simulink model "tb_gnc"  (R2026b)
settings: Solver=ode3  StopTime=10  FixedStep=1e-3  EnableMultiTasking=on
values from neighbouring files (symbols this model uses):
  P = F.P    [gnc_fsm_driver.m]    (also in t_gnc_mission.m = r.P; t_t07_gnc_sil.m = shaddad_params('World', 3, 'Assign', false))
  Ts = pr.Ts    [t_gnc_mission.m]
undefined symbols (not defined in the file or in its folder): aligned, DiscIntNeverNeededParam, drive_ready, eul, gnssFixType, headingValid, heartbeat, NavQuality, navValid, pos_W, posStd, power_ready, quality, rc_link_ok, rc_mode_sw, SOC, v_track_meas, valid, vel_B, yawRate
libraries: simulink x3, robotmobilelib x1
settings Model: Creator=aomar  LastModifiedBy=aomar
settings ConfigSet: Description=Shaddad fixed-step 1 ms ode3, multitasking, explicit rate transitions (arch 7, D58).
settings DataIOCC: SignalLogging=off
settings OptimizationCC: SimCompilerOptimization=on
settings DebuggingCC: AlgebraicLoopMsg=error  ArtificialAlgebraicLoopMsg=error  SingleTaskRateTransMsg=error  StrictBusMsg=ErrorOnBusTreatedAsVector
settings SimscapeCC: SimscapeNominalValues="[{\"value\":\"1\",\"unit\":\"A\"},{\"value\":\"1\",\"unit\":\"bar\"},{\"value\":\"1\",\"unit\":\"cm^2\"},{\"value\":\"1\",\"unit\":\"cm^3/s\"},{\"value\":\"1\",\"unit\":\"kJ/kg\"},{\"value\":\"1\",\"unit\":\"kW\"},{\"value\":\"1\",\"unit\":\"l\"},{\"value\":\"1\",\"unit\":\"N\"},{\"value\":\"1\",\"unit\":\"N*m\"},{\"value\":\"1\",\"unit\":\"V\"},{\"value\":\"0.001\",\"unit\":\"Wb\"}]"  SimscapeNormalizeSystem=off  SimscapeUseEnergyAccounting=off

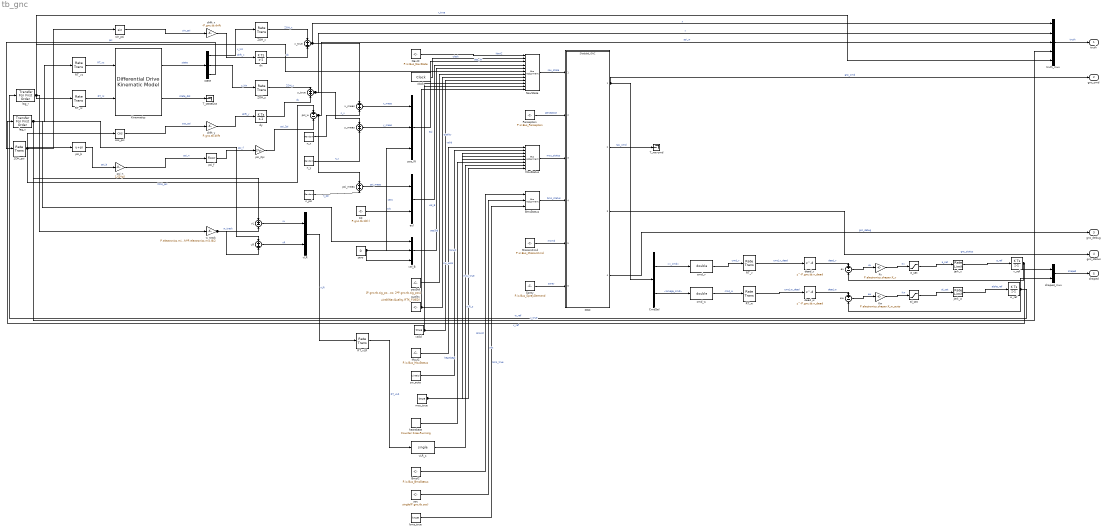
== system tb_gnc ==
  BmsIC : Constant  Value=P.ic.Bus_BmsStatus  OutDataTypeStr=Bus: Bus_BmsStatus  SampleTime=Ts.hk
  BmsStatus : BusAssignment  AssignedSignals=SOC,valid
  CmdSel : BusSelector  OutputSignals=v_cmd,omega_cmd
  GNC : ModelReference  ModelNameDialog=Shaddad_GNC  SimulationMode=Normal  ModelReferenceVersion=1.1
  Kinematics : robotmobilelib/Differential Drive Kinematic Model  VehicleInputs=Vehicle Speed & Heading Angular Velocity  WheelRadius=P.structure.r_sprocket  WheelSpeedRange=[-inf inf]  TrackWidth=P.structure.geom.B  InitialState=P.gnc.tb.x0(:)  SimulateUsing=Code generation
  Kv : Gain  Gain=P.electronics.shaper.K_v
  Kw : Gain  Gain=P.electronics.shaper.K_w_auto
  McuIC : Constant  Value=P.ic.Bus_McuStatus  OutDataTypeStr=Bus: Bus_McuStatus  SampleTime=Ts.gnc
  McuStatus : BusAssignment  AssignedSignals=rc_mode_sw,rc_link_ok,drive_ready,power_ready,heartbeat,v_track_meas,valid
  MissionCmd : Constant  Value=P.ic.Bus_MissionCmd  OutDataTypeStr=Bus: Bus_MissionCmd  SampleTime=Ts.mcmd
  NavIC : Constant  Value=P.ic.Bus_NavState  OutDataTypeStr=Bus: Bus_NavState  SampleTime=Ts.ctrl
  NavState : BusAssignment  AssignedSignals=t,pos_W,eul,vel_B,yawRate,posStd,quality,navValid,headingValid,aligned,gnssFixType
  Perception : Constant  Value=P.ic.Bus_Perception  OutDataTypeStr=Bus: Bus_Perception  SampleTime=Ts.perception
  RT_rc : RateTransition  OutPortSampleTime=0
  RT_v : RateTransition  OutPortSampleTime=Ts.ctrl
  RT_vLR : RateTransition  OutPortSampleTime=Ts.gnc
  RT_vc : RateTransition  OutPortSampleTime=0
  RT_w : RateTransition  OutPortSampleTime=Ts.ctrl
  Spray : Constant  Value=P.ic.Bus_SprayDemand  OutDataTypeStr=Bus: Bus_SprayDemand  SampleTime=Ts.spray
  T_navcmd : Terminator
  T_stateDot : Terminator
  ZOH_psi : RateTransition  OutPortSampleTime=Ts.ctrl
  ZOH_x : RateTransition  OutPortSampleTime=Ts.ctrl
  ZOH_y : RateTransition  OutPortSampleTime=Ts.ctrl
  a_sat : Saturate  UpperLimit=P.electronics.shaper.a_acc_auto  LowerLimit=-P.electronics.shaper.a_dec_auto
  al_sat : Saturate  UpperLimit=P.electronics.shaper.alpha_auto  LowerLimit=-P.electronics.shaper.alpha_auto
  bms_true : Constant  Value=true  OutDataTypeStr=boolean  SampleTime=Ts.hk
  clock : DigitalClock  SampleTime=Ts.ctrl
  cmd_v : DataTypeConversion  OutDataTypeStr=double  SaturateOnIntegerOverflow=off  RndMeth=Floor
  cmd_w : DataTypeConversion  OutDataTypeStr=double  SaturateOnIntegerOverflow=off  RndMeth=Floor
  cos_psi : Trigonometry  Operator=cos
  dead_v : Delay  DelayLength=P.gnc.tb.n_dead  InitialCondition=0  SampleTime=Ts.ctrl
  dead_w : Delay  DelayLength=P.gnc.tb.n_dead  InitialCondition=0  SampleTime=Ts.ctrl
  drift_x : Gain  Gain=-P.gnc.tb.drift
  drift_y : Gain  Gain=P.gnc.tb.drift
  dx : DiscreteIntegrator  SampleTime=Ts.ctrl  ICPrevOutput=DiscIntNeverNeededParam  ICPrevScaledInput=DiscIntNeverNeededParam
  dy : DiscreteIntegrator  SampleTime=Ts.ctrl  ICPrevOutput=DiscIntNeverNeededParam  ICPrevScaledInput=DiscIntNeverNeededParam
  eul : Mux  Inputs=[1 2]
  ev : Sum  Inputs=+-
  ew : Sum  Inputs=+-
  heartbeat : simulink/Sources/Counter Free-Running  NumBits=8  tsamp=Ts.gnc
  jerk_v : RateLimiter  RisingSlewLimit=P.electronics.shaper.j_max  FallingSlewLimit=-P.electronics.shaper.j_max  SampleTimeMode=inherited
  jerk_w : RateLimiter  RisingSlewLimit=P.electronics.shaper.jw_auto  FallingSlewLimit=-P.electronics.shaper.jw_auto  SampleTimeMode=inherited
  lag_r : simulink/Discrete/Transfer Fcn First Order  PoleZ=exp(-Ts.ctrl/P.gnc.tb.tau_r)  ICPrevOutput=0.0  DoSatur=off
  lag_v : simulink/Discrete/Transfer Fcn First Order  PoleZ=exp(-Ts.ctrl/P.gnc.tb.tau_v)  ICPrevOutput=0.0  DoSatur=off
  mcu_true : Constant  Value=true  OutDataTypeStr=boolean  SampleTime=Ts.gnc
  n_psi : RandomNumber  Variance=P.gnc.tb.sig_yaw^2  Seed=P.gnc.tb.seed_psi  SampleTime=Ts.ctrl
  n_x : RandomNumber  Variance=P.gnc.tb.sig_pos^2  Seed=P.gnc.tb.seed_x  SampleTime=Ts.ctrl
  n_y : RandomNumber  Variance=P.gnc.tb.sig_pos^2  Seed=P.gnc.tb.seed_y  SampleTime=Ts.ctrl
  posStd : Constant  Value=[P.gnc.tb.sig_pos; P.gnc.tb.sig_pos; 2*P.gnc.tb.sig_pos]  SampleTime=Ts.ctrl
  pos_W : Mux  Inputs=3
  psi_2pi : Gain  Gain=2*pi
  psi_b : Bias  Bias=pi  SaturateOnIntegerOverflow=off
  psi_f : Rounding
  psi_meas : Sum
  psi_n : Gain  Gain=1/(2*pi)
  psi_w : Sum  Inputs=+-
  quality : Constant  Value=uint8(NavQuality.RTK_FIXED)  OutDataTypeStr=uint8  SampleTime=Ts.ctrl
  shaped_mux : Mux  Inputs=2
  sin_psi : Trigonometry
  soc : Constant  Value=single(P.gnc.tb.soc)  OutDataTypeStr=single  SampleTime=Ts.hk
  state : Demux  Outputs=3
  sw_auto : Constant  Value=uint8(2)  OutDataTypeStr=uint8  SampleTime=Ts.gnc
  tilt : Constant  Value=P.gnc.tb.tilt(:)  SampleTime=Ts.ctrl
  truth_mux : Mux  Inputs=5
  vL : Sum  Inputs=+-
  vLR : Mux  Inputs=2
  vLR_s : DataTypeConversion  OutDataTypeStr=single  SaturateOnIntegerOverflow=off  RndMeth=Floor
  vR : Sum
  v_ref : DiscreteIntegrator  SampleTime=Ts.ctrl  ICPrevOutput=DiscIntNeverNeededParam  ICPrevScaledInput=DiscIntNeverNeededParam
  valid : Constant  Value=true  OutDataTypeStr=boolean  SampleTime=Ts.ctrl
  vel_B : Mux  Inputs=3
  w_ref : DiscreteIntegrator  SampleTime=Ts.ctrl  ICPrevOutput=DiscIntNeverNeededParam  ICPrevScaledInput=DiscIntNeverNeededParam
  w_track : Gain  Gain=P.electronics.mix.chi*P.electronics.mix.B/2
  x_meas : Sum
  x_true : Sum
  y_meas : Sum
  y_true : Sum
  zero : Constant  Value=0  SampleTime=Ts.ctrl
  truth : Outport
  gnc_cmd : Outport  Port=2
  gnc_debug : Outport  Port=3
  gnc_status : Outport  Port=4
  shaped : Outport  Port=5
  wires:
  ZOH_psi/1 -> sin_psi/1, psi_w/1, cos_psi/1, psi_b/1  "ZOH_psi"
  lag_v/1 -> vel_B/1, vR/1, vL/1, truth_mux/4, RT_vc/1  "v_true"
  lag_r/1 -> w_track/1, truth_mux/5, NavState/6, RT_rc/1  "r_true"
  RT_vc/1 -> Kinematics/1  "RT_vc"
  RT_rc/1 -> Kinematics/2  "RT_rc"
  psi_b/1 -> psi_n/1  "psi_b"
  sin_psi/1 -> drift_x/1  "sin_psi"
  cos_psi/1 -> drift_y/1  "cos_psi"
  psi_n/1 -> psi_f/1  "psi_n"
  Kinematics/1 -> state/1  "state"
  Kinematics/2 -> T_stateDot/1  "state_dot"
  state/1 -> ZOH_x/1  "x_kin"
  state/2 -> ZOH_y/1  "y_kin"
  state/3 -> ZOH_psi/1  "psi"
  drift_x/1 -> dx/1  "drift_x"
  drift_y/1 -> dy/1  "drift_y"
  psi_f/1 -> psi_2pi/1  "psi_f"
  w_track/1 -> vR/2, vL/2  "w_track"
  vL/1 -> vLR/1  "vL"
  vR/1 -> vLR/2  "vR"
  psi_2pi/1 -> psi_w/2  "psi_2pi"
  dx/1 -> x_true/2  "dx"
  dy/1 -> y_true/2  "dy"
  ZOH_x/1 -> x_true/1  "ZOH_x"
  ZOH_y/1 -> y_true/1  "ZOH_y"
  vLR/1 -> RT_vLR/1  "vLR"
  x_true/1 -> x_meas/1, truth_mux/1  "x"
  y_true/1 -> truth_mux/2, y_meas/1  "y"
  n_x/1 -> x_meas/2  "n_x"
  n_y/1 -> y_meas/2  "n_y"
  n_psi/1 -> psi_meas/2  "n_psi"
  psi_w/1 -> truth_mux/3, psi_meas/1  "psi_w"
  x_meas/1 -> pos_W/1  "x_meas"
  y_meas/1 -> pos_W/2  "y_meas"
  psi_meas/1 -> eul/1  "psi_meas"
  tilt/1 -> eul/2  "tilt"
  zero/1 -> pos_W/3, vel_B/3, vel_B/2  "zero"
  RT_vLR/1 -> vLR_s/1  "RT_vLR"
  pos_W/1 -> NavState/3  "pos_W"
  eul/1 -> NavState/4  "eul"
  vel_B/1 -> NavState/5  "vel_B"
  NavIC/1 -> NavState/1  "NavIC"
  posStd/1 -> NavState/7  "posStd"
  quality/1 -> NavState/8, NavState/12  "quality"
  McuIC/1 -> McuStatus/1  "McuIC"
  sw_auto/1 -> McuStatus/2  "sw_auto"
  heartbeat/1 -> McuStatus/6  "heartbeat"
  BmsIC/1 -> BmsStatus/1  "BmsIC"
  soc/1 -> BmsStatus/2  "soc"
  bms_true/1 -> BmsStatus/3  "bms_true"
  valid/1 -> NavState/9, NavState/10, NavState/11  "valid"
  mcu_true/1 -> McuStatus/3, McuStatus/4, McuStatus/5, McuStatus/8  "mcu_true"
  clock/1 -> NavState/2  "clock"
  vLR_s/1 -> McuStatus/7  "vLR_s"
  Perception/1 -> GNC/2  "perception"
  MissionCmd/1 -> GNC/5  "mcmd"
  Spray/1 -> GNC/6  "spray"
  NavState/1 -> GNC/1  "nav_state"
  McuStatus/1 -> GNC/3  "mcu_status"
  BmsStatus/1 -> GNC/4  "bms_status"
  GNC/1 -> CmdSel/1, gnc_cmd/1  "gnc_cmd"
  GNC/2 -> T_navcmd/1  "nav_cmd"
  GNC/3 -> gnc_status/1  "gnc_status"
  GNC/4 -> gnc_debug/1  "gnc_debug"
  CmdSel/1 -> cmd_v/1  "<v_cmd>"
  CmdSel/2 -> cmd_w/1  "<omega_cmd>"
  cmd_v/1 -> RT_v/1  "cmd_v"
  cmd_w/1 -> RT_w/1  "cmd_w"
  RT_v/1 -> dead_v/1  "cmd_v_dead"
  RT_w/1 -> dead_w/1  "cmd_w_dead"
  dead_v/1 -> ev/1  "dead_v"
  dead_w/1 -> ew/1  "dead_w"
  ev/1 -> Kv/1  "ev"
  ew/1 -> Kw/1  "ew"
  Kv/1 -> a_sat/1  "Kv"
  Kw/1 -> al_sat/1  "Kw"
  a_sat/1 -> jerk_v/1  "a_sat"
  al_sat/1 -> jerk_w/1  "al_sat"
  jerk_v/1 -> v_ref/1  "a_ref"
  jerk_w/1 -> w_ref/1  "alpha_ref"
  w_ref/1 -> lag_r/1, ew/2, shaped_mux/2  "w_ref"
  v_ref/1 -> lag_v/1, ev/2, shaped_mux/1  "v_ref"
  truth_mux/1 -> truth/1  "truth"
  shaped_mux/1 -> shaped/1  "shaped"
